simulink model "demoCS2passiveObserverDP"  (R2024a)
settings: Solver=ode45  StartTime=0.0  StopTime=200  RelTol=1e-3  EnableMultiTasking=on
libraries: mssSimulink x6, simulink_extras x4, simulink x2
settings Model: Creator=Thor  LastModifiedBy=thor
settings SolverCC: AlgebraicLoopSolver=TrustRegion
settings DataIOCC: LimitDataPoints=on  SaveFormat=Array  SignalLoggingSaveFormat=ModelDataLogs  ReturnWorkspaceOutputs=off  SignalLoggingName=sigsOut
settings OptimizationCC: ExpressionDepthLimit=2147483647  InitFltsAndDblsToZero=on  LifeSpan=inf
settings DebuggingCC: SaveWithParameterizedLinksMsg=none  UnderspecifiedInitializationDetection=Classic  MergeDetectMultiDrivingBlocksExec=none  SignalResolutionControl=TryResolveAllWithWarning  MultiTaskDSMMsg=warning  MultiTaskCondExecSysMsg=none  FcnCallInpInsideContextMsg=warning  UnconnectedInputMsg=warning  UnconnectedOutputMsg=warning  UnconnectedLineMsg=warning  StateNameClashWarn=warning  SFUnexpectedBacktrackingDiag=warning  SFNoUnconditionalDefaultTransitionDiag=warning  SFExecutionAtInitializationDiag=none  ArithmeticOperatorsInVariantConditions=warning
settings HardwareCC: ProdBitPerPointer=32  ProdBitPerSizeT=32  ProdBitPerPtrDiffT=32  ProdLargestAtomicFloat=None  ProdIntDivRoundTo=Undefined  ProdEndianess=Unspecified  ProdWordSize=32  ProdHWDeviceType=32-bit Generic  TargetUnknown=on
settings ModelReferenceCC: EnableRefExpFcnMdlSchedulingChecks=on  PropagateSignalLabelsOutOfModel=off
settings RTWCC: GPUComputeCapability=3.5  DLArmComputeVersion=19.05
settings CodeAppCC: StateflowObjectComments=on
settings GRTTargetCC: TargetFcnLib=ansi_tfl_tmw.mat  TargetLangStandard=C89/C90 (ANSI)  ModelReferenceCompliant=off  CombineOutputUpdateFcns=off  MatFileLogging=off  GRTInterface=on
settings ConfigComp: CovMetricSettings=dw  CovSaveCumulativeToWorkspaceVar=on  CovSaveSingleToWorkspaceVar=on

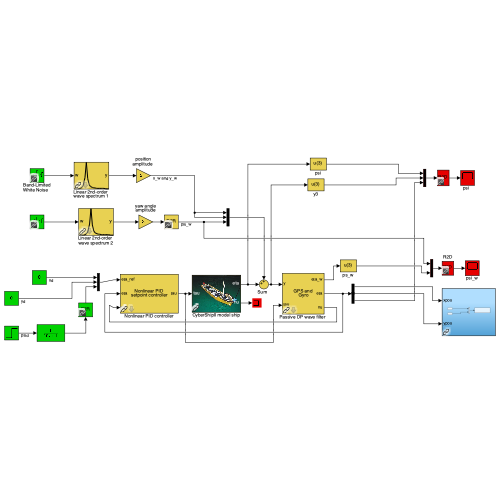
[thumbnail: Simulink's stored preview of the top-level diagram]
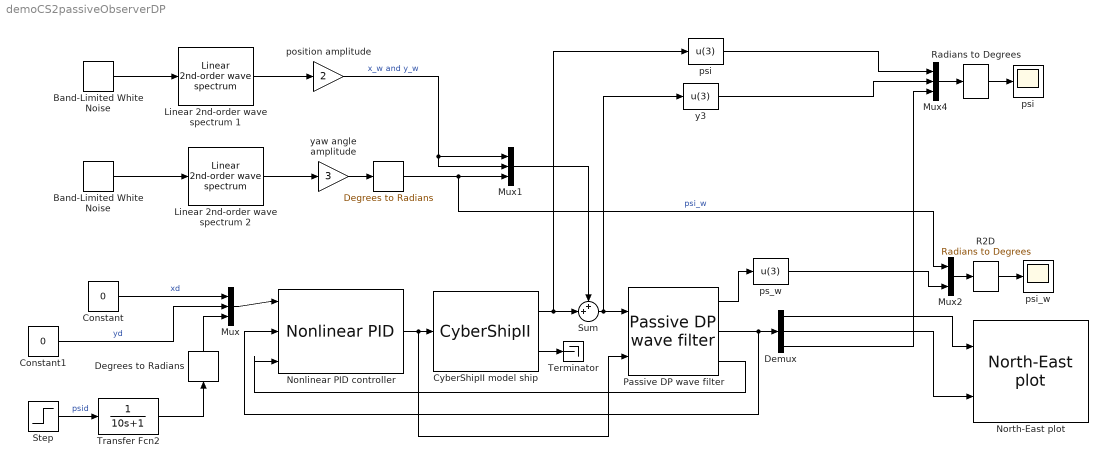
== system demoCS2passiveObserverDP ==
  "   " : simulink_extras/Transformations/Degrees to Radians
  Band-Limited White Noise : simulink/Sources/Band-Limited White Noise  Cov=[1]  Ts=0.1  seed=[23341]
  "Band-Limited White Noise  " : simulink/Sources/Band-Limited White Noise  Cov=[1]  Ts=0.1  seed=[23341]
  Constant : Constant  Value=0
  Constant1 : Constant  Value=0
  CyberShipII model ship : mssSimulink/Marine craft models/CyberShipII  SystemSampleTime=-1  VariantActivationTime=update diagram  AllowFlexibleInterface=on  Latency=0  AutoFrameSizeCalculation=off
  Degrees to Radians : simulink_extras/Transformations/Degrees to Radians
  Demux : Demux  Outputs=3
      settings: DisplayOption=none
  Linear 2nd-order wave spectrum 1 : mssSimulink/Environment/Waves/Linear 2nd-order  wave spectrum  sigma=0.5  w_0=0.8  lambda=0.1
  Linear 2nd-order wave spectrum 2 : mssSimulink/Environment/Waves/Linear 2nd-order  wave spectrum  sigma=0.5  w_0=0.8  lambda=0.1
  Mux : Mux  Inputs=3
  Mux1 : Mux  Inputs=3
  Mux2 : Mux  Inputs=2
  Mux4 : Mux  Inputs=3
  Nonlinear PID controller : mssSimulink/Control/DP/Nonlinear PID  Kp="(0.1)^2*[25.8000 0  0;  0  33.8000  1.0115;  0  1.0115  2.7600 ]"  Kd="2*0.8*0.1*[25.8000 0  0;  0  33.8000  1.0115;  0  1.0115  2.7600 ]"  Ki="(0.1^3/10)*[25.8000 0  0;  0  33.8000  1.0115;  0  1.0115  2.7600 ]"
  "North-East plot  " : mssSimulink/Utilities/Visualization/North-East plot    SystemSampleTime=-1  VariantActivationTime=update diagram  AllowFlexibleInterface=on  Latency=0  AutoFrameSizeCalculation=off
  "Passive DP wave filter " : mssSimulink/Navigation/Estimators/Passive DP wave filter  lambda=0.1*diag([1 1 1])  w_o=diag([0.8 0.8 0.8])  K4=0.1*diag([1 1 0.1])  K3=0.1*diag([1 1 0.1])  w_c=1.3*diag([0.8 0.8 0.8])  T_b=diag([100 100 100])  M="[ 25.8000   0    0;   0   33.8000   1.0115; 0   1.0115    2.7600 ]"  D="[2 0  0;  0 7 0.1; 0 0.1 0.5]"
  R2D : simulink_extras/Transformations/Radians to Degrees
  Radians to Degrees : simulink_extras/Transformations/Radians to Degrees
  Step : Step  Time=30  After=10  SampleTime=0
  "Sum  " : Sum  Inputs=++|  InputSameDT=on  SaturateOnIntegerOverflow=on  OutDataTypeStr=Inherit: Same as first input
  Terminator : Terminator
  Transfer Fcn2 : TransferFcn  Denominator=[10 1]
  "position amplitude " : Gain  Gain=2  SaturateOnIntegerOverflow=on  OutDataTypeStr=Inherit: Same as input  ParamDataTypeStr=Inherit: Same as input
  ps_w : Fcn  Expr=u(3)
  psi : Fcn  Expr=u(3)
  "psi  " : Scope
  psi_w : Scope
  y3 : Fcn  Expr=u(3)
  yaw angle amplitude : Gain  Gain=3  SaturateOnIntegerOverflow=on  OutDataTypeStr=Inherit: Same as input  ParamDataTypeStr=Inherit: Same as input
  wires:
  Constant/1 -> Mux/1  "xd"
  Step/1 -> Transfer Fcn2/1  "psid"
  Degrees to Radians/1 -> Mux/3
  Constant1/1 -> Mux/2  "yd"
  Demux/1 -> "North-East plot  "/1
  Demux/2 -> "North-East plot  "/2
  Mux/1 -> Nonlinear PID controller/1
  Transfer Fcn2/1 -> Degrees to Radians/1
  Band-Limited White Noise/1 -> Linear 2nd-order wave spectrum 2/1
  Linear 2nd-order wave spectrum 2/1 -> yaw angle amplitude/1
  yaw angle amplitude/1 -> "   "/1
  "Band-Limited White Noise  "/1 -> Linear 2nd-order wave spectrum 1/1
  Linear 2nd-order wave spectrum 1/1 -> "position amplitude "/1
  "position amplitude "/1 -> Mux1/2, Mux1/1  "x_w and y_w"
  "   "/1 -> Mux1/3, Mux2/1  "psi_w"
  Mux1/1 -> "Sum  "/1
  CyberShipII model ship/1 -> "Sum  "/2, psi/1
  Mux2/1 -> R2D/1
  "Sum  "/1 -> y3/1, "Passive DP wave filter "/1
  Radians to Degrees/1 -> "psi  "/1
  CyberShipII model ship/2 -> Terminator/1
  R2D/1 -> psi_w/1
  ps_w/1 -> Mux2/2
  Mux4/1 -> Radians to Degrees/1
  Demux/3 -> Mux4/3
  y3/1 -> Mux4/2
  psi/1 -> Mux4/1
  "Passive DP wave filter "/2 -> Demux/1, Nonlinear PID controller/2
  "Passive DP wave filter "/1 -> ps_w/1
  Nonlinear PID controller/1 -> "Passive DP wave filter "/2, CyberShipII model ship/1
  "Passive DP wave filter "/3 -> Nonlinear PID controller/3
